simulink model "pam3_patent_demo"  (R2022a)
settings: Solver=FixedStepDiscrete  StartTime=0  StopTime=pam3_stop_time  FixedStep=pam3_cfg.sample_time  RelTol=1e-3
undefined symbols (not defined in the file): pam3_cfg
Description:
  | Structurally authored model. Rebuild via build_pam3_models in MATLAB; Simulink execution pending.
settings SolverCC: AlgebraicLoopSolver=TrustRegion
settings DataIOCC: SaveOutput=off  SignalLogging=off  SaveTime=off
settings OptimizationCC: LifeSpan=inf
settings DebuggingCC: UnconnectedInputMsg=warning  UnconnectedOutputMsg=warning  UnconnectedLineMsg=warning  SFMachineParentedDataDiag=warning  ArithmeticOperatorsInVariantConditions=warning
settings SFSimCC: SimUseLocalCustomCode=off  CustomCodeUndefinedFunction=UseInterfaceOnly
settings RTWCC: RTWUseLocalCustomCode=off  DLArmComputeVersion=19.05
settings CodeAppCC: StateflowObjectComments=on

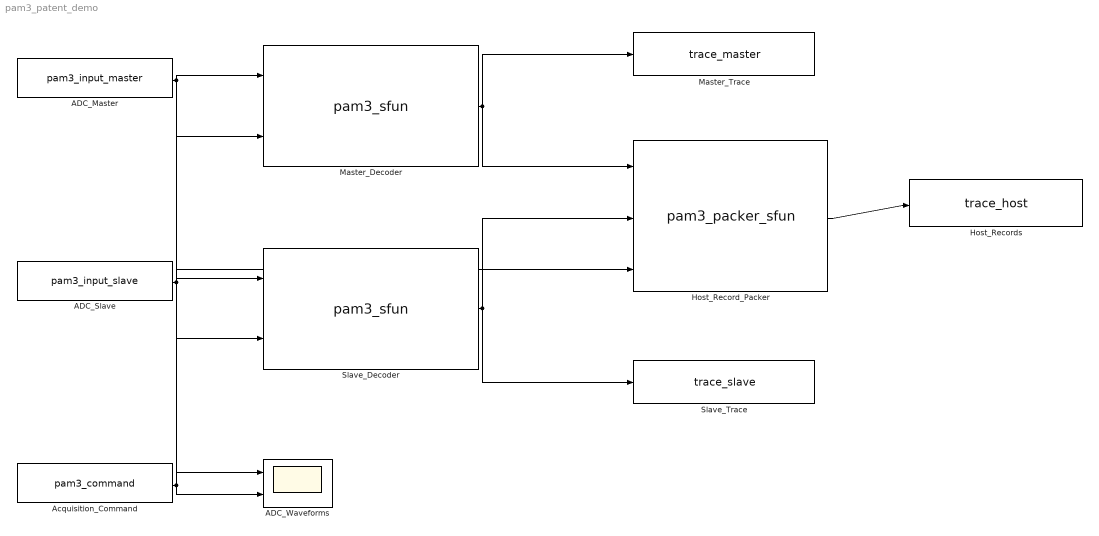
== system pam3_patent_demo ==
  ADC_Master : FromWorkspace  VariableName=pam3_input_master  SampleTime=pam3_cfg.sample_time  Interpolate=off  OutputAfterFinalValue=Holding final value
  ADC_Slave : FromWorkspace  VariableName=pam3_input_slave  SampleTime=pam3_cfg.sample_time  Interpolate=off  OutputAfterFinalValue=Holding final value
  Acquisition_Command : FromWorkspace  VariableName=pam3_command  SampleTime=pam3_cfg.sample_time  Interpolate=off  OutputAfterFinalValue=Holding final value
  Master_Decoder : M-S-Function  FunctionName=pam3_sfun  Parameters=pam3_cfg  DisplayMFileStacktrace=on
  Slave_Decoder : M-S-Function  FunctionName=pam3_sfun  Parameters=pam3_cfg  DisplayMFileStacktrace=on
  Host_Record_Packer : M-S-Function  FunctionName=pam3_packer_sfun  Parameters=pam3_cfg  DisplayMFileStacktrace=on
  Master_Trace : ToWorkspace  VariableName=trace_master  SaveFormat=Structure With Time  SampleTime=-1
  Slave_Trace : ToWorkspace  VariableName=trace_slave  SaveFormat=Structure With Time  SampleTime=-1
  Host_Records : ToWorkspace  VariableName=trace_host  SaveFormat=Structure With Time  SampleTime=-1
  ADC_Waveforms : Scope  NumInputPorts=2
  wires:
  ADC_Master/1 -> Master_Decoder/1, ADC_Waveforms/1
  ADC_Slave/1 -> Slave_Decoder/1, ADC_Waveforms/2
  Acquisition_Command/1 -> Master_Decoder/2, Slave_Decoder/2, Host_Record_Packer/3
  Master_Decoder/1 -> Master_Trace/1, Host_Record_Packer/1
  Slave_Decoder/1 -> Slave_Trace/1, Host_Record_Packer/2
  Host_Record_Packer/1 -> Host_Records/1
